simulink model "afe_dq_ttype"  (R2026b)
settings: Solver=ode23tb  StopTime=param.sim.simlength  FixedStep=param.sim.tc  MaxStep=param.glb_time.tc
values from neighbouring files (symbols this model uses):
  param = struct()    [init_model.m]
undefined symbols (not defined in the file or in its folder): magnitude
libraries: fl_lib x281, nesl_utility x136, igbt_simple_2th_lib x12, single_phase_transformer_lib x3, discrete_time_low_pass_filter x1, threephase_inductor_lib x1, dclink_for_three_levels x1, three_phase_three_level_ttype_inverter_ideal_switch_based_model x1, three_phase_three_levels_PWM_modulator x1, three_phase_bridge_three_level_ttype_igbt_simple_2th x1, three_phase_voltage_with_frt_emulator_mfcn x1
(part 4 of 8)

== system afe_dq_ttype/afe_dq_mod1/afe/deadtime_generator_for_ttype/dead_time_generator_cmos_simulink_phv/dead_time_leg_generator_1 ==
  cmd_in_QA : Inport
  cmd_in_QB : Inport  Port=2
  MATLAB Function : MATLAB Function  TreatAsAtomicUnit=on
  MATLAB Function1 : MATLAB Function  TreatAsAtomicUnit=on
  MATLAB Function2 : MATLAB Function  TreatAsAtomicUnit=on
  MATLAB Function3 : MATLAB Function  TreatAsAtomicUnit=on
  MATLAB Function4 : MATLAB Function  TreatAsAtomicUnit=on
  MATLAB Function5 : MATLAB Function  TreatAsAtomicUnit=on
  MATLAB Function6 : MATLAB Function  TreatAsAtomicUnit=on
  MATLAB Function7 : MATLAB Function  TreatAsAtomicUnit=on
  MATLAB Function8 : MATLAB Function  TreatAsAtomicUnit=on
  MATLAB Function9 : MATLAB Function  TreatAsAtomicUnit=on
  Transfer Fcn : TransferFcn  Denominator=[sqrt(2)*deadtime 1]
  Transfer Fcn1 : TransferFcn  Denominator=[sqrt(2)*deadtime 1]
  cmd_out_QA : Outport
  cmd_out_QB : Outport  Port=2
  wires:
  Transfer Fcn/1 -> MATLAB Function3/1(u)
  Transfer Fcn1/1 -> MATLAB Function8/1(u)
  cmd_in_QB/1 -> MATLAB Function6/1(u)
  MATLAB Function1/1(y) -> MATLAB Function9/1(u1)
  MATLAB Function5/1(y) -> MATLAB Function4/2(u2)
  cmd_in_QA/1 -> MATLAB Function/1(u)
  MATLAB Function6/1(y) -> MATLAB Function7/1(u), MATLAB Function5/1(u1)
  MATLAB Function4/1(y) -> cmd_out_QA/1
  MATLAB Function9/1(y) -> cmd_out_QB/1
  MATLAB Function/1(y) -> MATLAB Function2/1(u), MATLAB Function1/1(u1)
  MATLAB Function2/1(y) -> MATLAB Function4/1(u1), Transfer Fcn/1
  MATLAB Function3/1(y) -> MATLAB Function1/2(u2)
  MATLAB Function7/1(y) -> MATLAB Function9/2(u2), Transfer Fcn1/1
  MATLAB Function8/1(y) -> MATLAB Function5/2(u2)

== system afe_dq_ttype/afe_dq_mod1/afe/deadtime_generator_for_ttype/dead_time_generator_cmos_simulink_phw/dead_time_leg_generator_1 ==
  cmd_in_QA : Inport
  cmd_in_QB : Inport  Port=2
  MATLAB Function : MATLAB Function  TreatAsAtomicUnit=on
  MATLAB Function1 : MATLAB Function  TreatAsAtomicUnit=on
  MATLAB Function2 : MATLAB Function  TreatAsAtomicUnit=on
  MATLAB Function3 : MATLAB Function  TreatAsAtomicUnit=on
  MATLAB Function4 : MATLAB Function  TreatAsAtomicUnit=on
  MATLAB Function5 : MATLAB Function  TreatAsAtomicUnit=on
  MATLAB Function6 : MATLAB Function  TreatAsAtomicUnit=on
  MATLAB Function7 : MATLAB Function  TreatAsAtomicUnit=on
  MATLAB Function8 : MATLAB Function  TreatAsAtomicUnit=on
  MATLAB Function9 : MATLAB Function  TreatAsAtomicUnit=on
  Transfer Fcn : TransferFcn  Denominator=[sqrt(2)*deadtime 1]
  Transfer Fcn1 : TransferFcn  Denominator=[sqrt(2)*deadtime 1]
  cmd_out_QA : Outport
  cmd_out_QB : Outport  Port=2
  wires:
  MATLAB Function8/1(y) -> MATLAB Function5/2(u2)
  MATLAB Function7/1(y) -> Transfer Fcn1/1, MATLAB Function9/2(u2)
  MATLAB Function3/1(y) -> MATLAB Function1/2(u2)
  MATLAB Function2/1(y) -> Transfer Fcn/1, MATLAB Function4/1(u1)
  MATLAB Function/1(y) -> MATLAB Function1/1(u1), MATLAB Function2/1(u)
  MATLAB Function9/1(y) -> cmd_out_QB/1
  MATLAB Function4/1(y) -> cmd_out_QA/1
  MATLAB Function6/1(y) -> MATLAB Function5/1(u1), MATLAB Function7/1(u)
  cmd_in_QA/1 -> MATLAB Function/1(u)
  MATLAB Function5/1(y) -> MATLAB Function4/2(u2)
  MATLAB Function1/1(y) -> MATLAB Function9/1(u1)
  cmd_in_QB/1 -> MATLAB Function6/1(u)
  Transfer Fcn1/1 -> MATLAB Function8/1(u)
  Transfer Fcn/1 -> MATLAB Function3/1(u)

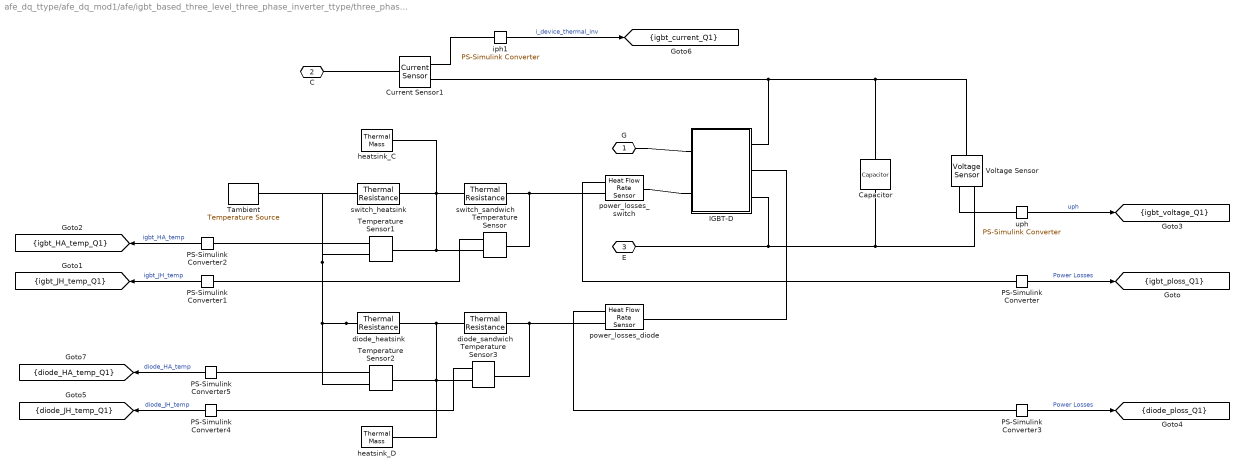
== system afe_dq_ttype/afe_dq_mod1/afe/igbt_based_three_level_three_phase_inverter_ttype/three_phase_inverter_igbt_2th_based_ttype/igbt_thermal_1 ==
  Capacitor : fl_lib/Electrical/Electrical Elements/Capacitor  c=Csnubber_m F  r=Rsnubber_m Ohm  g=0 1/Ohm  i_specify=off  i_priority=None  i=0 A  i_nominal_specify=off  i_nominal_value=1  i_nominal_unit=A  v_specify=off  v_priority=None  v=0 V  v_nominal_specify=off  v_nominal_value=1  v_nominal_unit=V  vc_specify=off  vc_priority=High  vc=0 V  vc_nominal_specify=off  vc_nominal_value=1  vc_nominal_unit=V
  Current Sensor1 : fl_lib/Electrical/Electrical Sensors/Current Sensor
  IGBT-D : Subsystem
  PS-Simulink Converter : nesl_utility/PS-Simulink Converter  PhysicalDomain=network_engine_domain  SubClassName=ps_output  LeftPortType=input  RightPortType=output  PseudoPeriodic=off  Frequencies=[]  VectorFormat=1-D array  Unit=W  AffineConversion=off
  PS-Simulink Converter{1..2,4..5} (4 alike) : nesl_utility/PS-Simulink Converter  PhysicalDomain=network_engine_domain  SubClassName=ps_output  LeftPortType=input  RightPortType=output  PseudoPeriodic=off  Frequencies=[]  VectorFormat=1-D array  Unit=degC  AffineConversion=off
  PS-Simulink Converter3 : nesl_utility/PS-Simulink Converter  PhysicalDomain=network_engine_domain  SubClassName=ps_output  LeftPortType=input  RightPortType=output  PseudoPeriodic=off  Frequencies=[]  VectorFormat=1-D array  Unit=W  AffineConversion=off
  Tambient : fl_lib/Thermal/Thermal Sources/Temperature Source  temperature=Tambient_m degC
  Temperature Sensor{,1..3} (4 alike) : fl_lib/Thermal/Thermal Sensors/Temperature Sensor  temperature_measure=foundation.enum.MeasurementReference.difference
  Voltage Sensor : fl_lib/Electrical/Electrical Sensors/Voltage Sensor
  diode_heatsink : fl_lib/Thermal/Thermal Elements/Thermal Resistance  resistance=rth_diode_HA_m K/W  T_specify=off  T_priority=High  T=0 deltadegC  T_nominal_specify=off  T_nominal_value=1  T_nominal_unit=K  Q_specify=off  Q_priority=None  Q=0 W  Q_nominal_specify=off  Q_nominal_value=1  Q_nominal_unit=W
  diode_sandwich : fl_lib/Thermal/Thermal Elements/Thermal Resistance  resistance=rth_diode_JH_m K/W  T_specify=off  T_priority=High  T=0 degC  T_nominal_specify=off  T_nominal_value=1  T_nominal_unit=K  Q_specify=off  Q_priority=None  Q=0 W  Q_nominal_specify=off  Q_nominal_value=1  Q_nominal_unit=W
  heatsink_C : fl_lib/Thermal/Thermal Elements/Thermal Mass  mass_type=foundation.enum.constant_variable.constant  mass=mass_heatsink_m kg  sp_heat=specific_heat_m J/(K*kg)  mass_min=1e-6 kg  num_ports=foundation.enum.numPorts2.one  m_specify=off  m_priority=High  m=1 kg  m_nominal_specify=off  m_nominal_value=1  m_nominal_unit=kg  T_specify=on  T_priority=High  T=DThs_init_m+Tambient_m degC  T_nominal_specify=off  T_nominal_value=1  T_nominal_unit=K  Q_specify=off  Q_priority=High  Q=0 W  Q_nominal_specify=off  Q_nominal_value=1  Q_nominal_unit=W
  heatsink_D : fl_lib/Thermal/Thermal Elements/Thermal Mass  mass_type=foundation.enum.constant_variable.constant  mass=mass_heatsink_m kg  sp_heat=specific_heat_m J/(K*kg)  mass_min=1e-6 kg  num_ports=foundation.enum.numPorts2.one  m_specify=off  m_priority=High  m=1 kg  m_nominal_specify=off  m_nominal_value=1  m_nominal_unit=kg  T_specify=on  T_priority=High  T=DThs_init_m+Tambient_m degC  T_nominal_specify=off  T_nominal_value=1  T_nominal_unit=K  Q_specify=off  Q_priority=High  Q=0 W  Q_nominal_specify=off  Q_nominal_value=1  Q_nominal_unit=W
  iph1 : nesl_utility/PS-Simulink Converter  PhysicalDomain=network_engine_domain  SubClassName=ps_output  LeftPortType=input  RightPortType=output  PseudoPeriodic=off  Frequencies=[]  VectorFormat=1-D array  Unit=A  AffineConversion=off
  power_losses_diode : fl_lib/Thermal/Thermal Sensors/Heat Flow Rate Sensor
  power_losses_switch : fl_lib/Thermal/Thermal Sensors/Heat Flow Rate Sensor
  switch_heatsink : fl_lib/Thermal/Thermal Elements/Thermal Resistance  resistance=rth_switch_HA_m K/W  T_specify=off  T_priority=High  T=0 deltadegC  T_nominal_specify=off  T_nominal_value=1  T_nominal_unit=K  Q_specify=off  Q_priority=None  Q=0 W  Q_nominal_specify=off  Q_nominal_value=1  Q_nominal_unit=W
  switch_sandwich : fl_lib/Thermal/Thermal Elements/Thermal Resistance  resistance=rth_switch_JH_m K/W  T_specify=off  T_priority=High  T=0 degC  T_nominal_specify=off  T_nominal_value=1  T_nominal_unit=K  Q_specify=off  Q_priority=None  Q=0 W  Q_nominal_specify=off  Q_nominal_value=1  Q_nominal_unit=W
  uph : nesl_utility/PS-Simulink Converter  PhysicalDomain=network_engine_domain  SubClassName=ps_output  LeftPortType=input  RightPortType=output  PseudoPeriodic=off  Frequencies=[]  VectorFormat=1-D array  Unit=V  AffineConversion=off
  G : PMIOPort  Side=Left
  C : PMIOPort  Port=2  Side=Left
  E : PMIOPort  Port=3  Side=Right
  tag scope: diode_HA_temp_Q1=scoped, diode_JH_temp_Q1=scoped, diode_ploss_Q1=scoped, igbt_HA_temp_Q1=scoped, igbt_JH_temp_Q1=scoped, igbt_current_Q1=scoped, igbt_ploss_Q1=scoped, igbt_voltage_Q1=scoped
  wires:
  PS-Simulink Converter/1 -> [igbt_ploss_Q1]  "Power Losses"
  PS-Simulink Converter2/1 -> [igbt_HA_temp_Q1]  "igbt_HA_temp"
  PS-Simulink Converter1/1 -> [igbt_JH_temp_Q1]  "igbt_JH_temp"
  iph1/1 -> [igbt_current_Q1]  "i_device_thermal_inv"
  uph/1 -> [igbt_voltage_Q1]  "uph"
  PS-Simulink Converter3/1 -> [diode_ploss_Q1]  "Power Losses"
  PS-Simulink Converter4/1 -> [diode_JH_temp_Q1]  "diode_JH_temp"
  PS-Simulink Converter5/1 -> [diode_HA_temp_Q1]  "diode_HA_temp"
  connections:
  Voltage Sensor/RConn2 -- Capacitor/RConn1 -- E/RConn1 -- IGBT-D/RConn3
  PS-Simulink Converter/LConn1 -- power_losses_switch/RConn1
  Temperature Sensor/LConn1 -- power_losses_switch/RConn2 -- switch_sandwich/LConn1
  Temperature Sensor1/LConn1 -- Temperature Sensor/RConn1 -- switch_sandwich/RConn1 -- switch_heatsink/LConn1 -- heatsink_C/LConn1
  Temperature Sensor/RConn2 -- PS-Simulink Converter1/LConn1
  diode_heatsink/RConn1 -- Temperature Sensor2/RConn1 -- Temperature Sensor1/RConn1 -- Tambient/LConn1 -- switch_heatsink/RConn1
  Temperature Sensor1/RConn2 -- PS-Simulink Converter2/LConn1
  Current Sensor1/LConn1 -- C/RConn1
  Capacitor/LConn1 -- Voltage Sensor/LConn1 -- Current Sensor1/RConn2 -- IGBT-D/RConn1
  Current Sensor1/RConn1 -- iph1/LConn1
  Voltage Sensor/RConn1 -- uph/LConn1
  power_losses_diode/RConn2 -- Temperature Sensor3/LConn1 -- diode_sandwich/LConn1
  heatsink_D/LConn1 -- Temperature Sensor2/LConn1 -- Temperature Sensor3/RConn1 -- diode_sandwich/RConn1 -- diode_heatsink/LConn1
  power_losses_diode/RConn1 -- PS-Simulink Converter3/LConn1
  Temperature Sensor2/RConn2 -- PS-Simulink Converter5/LConn1
  Temperature Sensor3/RConn2 -- PS-Simulink Converter4/LConn1
  IGBT-D/LConn2 -- power_losses_switch/LConn1
  G/RConn1 -- IGBT-D/LConn1
  IGBT-D/RConn2 -- power_losses_diode/LConn1

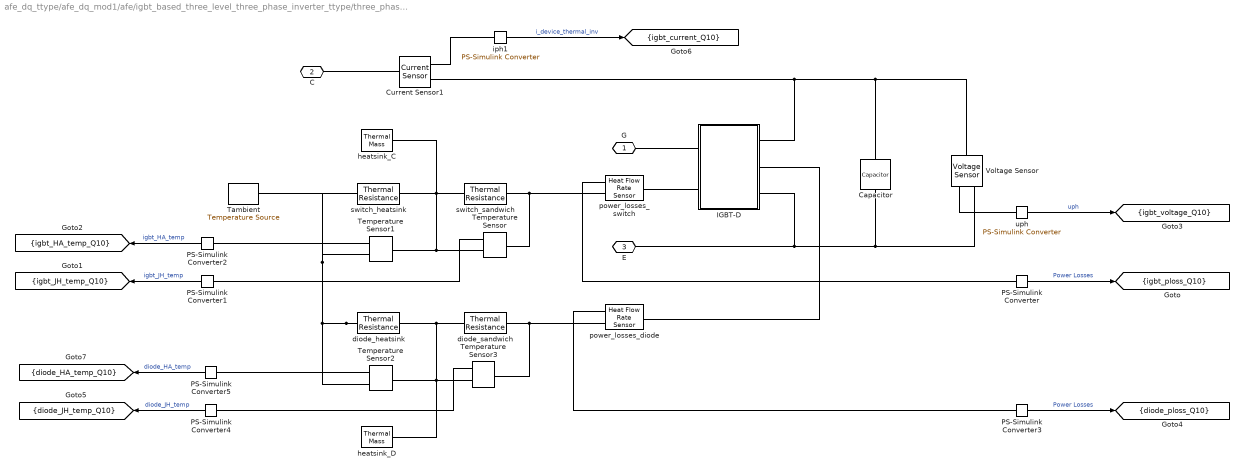
== system afe_dq_ttype/afe_dq_mod1/afe/igbt_based_three_level_three_phase_inverter_ttype/three_phase_inverter_igbt_2th_based_ttype/igbt_thermal_10 ==
  Capacitor : fl_lib/Electrical/Electrical Elements/Capacitor  c=Csnubber_m F  r=Rsnubber_m Ohm  g=0 1/Ohm  i_specify=off  i_priority=None  i=0 A  i_nominal_specify=off  i_nominal_value=1  i_nominal_unit=A  v_specify=off  v_priority=None  v=0 V  v_nominal_specify=off  v_nominal_value=1  v_nominal_unit=V  vc_specify=off  vc_priority=High  vc=0 V  vc_nominal_specify=off  vc_nominal_value=1  vc_nominal_unit=V
  Current Sensor1 : fl_lib/Electrical/Electrical Sensors/Current Sensor
  IGBT-D : Subsystem
  PS-Simulink Converter : nesl_utility/PS-Simulink Converter  PhysicalDomain=network_engine_domain  SubClassName=ps_output  LeftPortType=input  RightPortType=output  PseudoPeriodic=off  Frequencies=[]  VectorFormat=1-D array  Unit=W  AffineConversion=off
  PS-Simulink Converter{1..2,4..5} (4 alike) : nesl_utility/PS-Simulink Converter  PhysicalDomain=network_engine_domain  SubClassName=ps_output  LeftPortType=input  RightPortType=output  PseudoPeriodic=off  Frequencies=[]  VectorFormat=1-D array  Unit=degC  AffineConversion=off
  PS-Simulink Converter3 : nesl_utility/PS-Simulink Converter  PhysicalDomain=network_engine_domain  SubClassName=ps_output  LeftPortType=input  RightPortType=output  PseudoPeriodic=off  Frequencies=[]  VectorFormat=1-D array  Unit=W  AffineConversion=off
  Tambient : fl_lib/Thermal/Thermal Sources/Temperature Source  temperature=Tambient_m degC
  Temperature Sensor{,1..3} (4 alike) : fl_lib/Thermal/Thermal Sensors/Temperature Sensor  temperature_measure=foundation.enum.MeasurementReference.difference
  Voltage Sensor : fl_lib/Electrical/Electrical Sensors/Voltage Sensor
  diode_heatsink : fl_lib/Thermal/Thermal Elements/Thermal Resistance  resistance=rth_diode_HA_m K/W  T_specify=off  T_priority=High  T=0 deltadegC  T_nominal_specify=off  T_nominal_value=1  T_nominal_unit=K  Q_specify=off  Q_priority=None  Q=0 W  Q_nominal_specify=off  Q_nominal_value=1  Q_nominal_unit=W
  diode_sandwich : fl_lib/Thermal/Thermal Elements/Thermal Resistance  resistance=rth_diode_JH_m K/W  T_specify=off  T_priority=High  T=0 degC  T_nominal_specify=off  T_nominal_value=1  T_nominal_unit=K  Q_specify=off  Q_priority=None  Q=0 W  Q_nominal_specify=off  Q_nominal_value=1  Q_nominal_unit=W
  heatsink_C : fl_lib/Thermal/Thermal Elements/Thermal Mass  mass_type=foundation.enum.constant_variable.constant  mass=mass_heatsink_m kg  sp_heat=specific_heat_m J/(K*kg)  mass_min=1e-6 kg  num_ports=foundation.enum.numPorts2.one  m_specify=off  m_priority=High  m=1 kg  m_nominal_specify=off  m_nominal_value=1  m_nominal_unit=kg  T_specify=on  T_priority=High  T=DThs_init_m+Tambient_m degC  T_nominal_specify=off  T_nominal_value=1  T_nominal_unit=K  Q_specify=off  Q_priority=High  Q=0 W  Q_nominal_specify=off  Q_nominal_value=1  Q_nominal_unit=W
  heatsink_D : fl_lib/Thermal/Thermal Elements/Thermal Mass  mass_type=foundation.enum.constant_variable.constant  mass=mass_heatsink_m kg  sp_heat=specific_heat_m J/(K*kg)  mass_min=1e-6 kg  num_ports=foundation.enum.numPorts2.one  m_specify=off  m_priority=High  m=1 kg  m_nominal_specify=off  m_nominal_value=1  m_nominal_unit=kg  T_specify=on  T_priority=High  T=DThs_init_m+Tambient_m degC  T_nominal_specify=off  T_nominal_value=1  T_nominal_unit=K  Q_specify=off  Q_priority=High  Q=0 W  Q_nominal_specify=off  Q_nominal_value=1  Q_nominal_unit=W
  iph1 : nesl_utility/PS-Simulink Converter  PhysicalDomain=network_engine_domain  SubClassName=ps_output  LeftPortType=input  RightPortType=output  PseudoPeriodic=off  Frequencies=[]  VectorFormat=1-D array  Unit=A  AffineConversion=off
  power_losses_diode : fl_lib/Thermal/Thermal Sensors/Heat Flow Rate Sensor
  power_losses_switch : fl_lib/Thermal/Thermal Sensors/Heat Flow Rate Sensor
  switch_heatsink : fl_lib/Thermal/Thermal Elements/Thermal Resistance  resistance=rth_switch_HA_m K/W  T_specify=off  T_priority=High  T=0 deltadegC  T_nominal_specify=off  T_nominal_value=1  T_nominal_unit=K  Q_specify=off  Q_priority=None  Q=0 W  Q_nominal_specify=off  Q_nominal_value=1  Q_nominal_unit=W
  switch_sandwich : fl_lib/Thermal/Thermal Elements/Thermal Resistance  resistance=rth_switch_JH_m K/W  T_specify=off  T_priority=High  T=0 degC  T_nominal_specify=off  T_nominal_value=1  T_nominal_unit=K  Q_specify=off  Q_priority=None  Q=0 W  Q_nominal_specify=off  Q_nominal_value=1  Q_nominal_unit=W
  uph : nesl_utility/PS-Simulink Converter  PhysicalDomain=network_engine_domain  SubClassName=ps_output  LeftPortType=input  RightPortType=output  PseudoPeriodic=off  Frequencies=[]  VectorFormat=1-D array  Unit=V  AffineConversion=off
  G : PMIOPort  Side=Left
  C : PMIOPort  Port=2  Side=Left
  E : PMIOPort  Port=3  Side=Right
  tag scope: diode_HA_temp_Q10=scoped, diode_JH_temp_Q10=scoped, diode_ploss_Q10=scoped, igbt_HA_temp_Q10=scoped, igbt_JH_temp_Q10=scoped, igbt_current_Q10=scoped, igbt_ploss_Q10=scoped, igbt_voltage_Q10=scoped
  wires:
  PS-Simulink Converter/1 -> [igbt_ploss_Q10]  "Power Losses"
  PS-Simulink Converter2/1 -> [igbt_HA_temp_Q10]  "igbt_HA_temp"
  PS-Simulink Converter1/1 -> [igbt_JH_temp_Q10]  "igbt_JH_temp"
  iph1/1 -> [igbt_current_Q10]  "i_device_thermal_inv"
  uph/1 -> [igbt_voltage_Q10]  "uph"
  PS-Simulink Converter3/1 -> [diode_ploss_Q10]  "Power Losses"
  PS-Simulink Converter4/1 -> [diode_JH_temp_Q10]  "diode_JH_temp"
  PS-Simulink Converter5/1 -> [diode_HA_temp_Q10]  "diode_HA_temp"
  connections:
  Voltage Sensor/RConn2 -- Capacitor/RConn1 -- IGBT-D/RConn3 -- E/RConn1
  PS-Simulink Converter/LConn1 -- power_losses_switch/RConn1
  Temperature Sensor/LConn1 -- power_losses_switch/RConn2 -- switch_sandwich/LConn1
  Temperature Sensor1/LConn1 -- Temperature Sensor/RConn1 -- switch_sandwich/RConn1 -- switch_heatsink/LConn1 -- heatsink_C/LConn1
  Temperature Sensor/RConn2 -- PS-Simulink Converter1/LConn1
  diode_heatsink/RConn1 -- Temperature Sensor2/RConn1 -- Temperature Sensor1/RConn1 -- Tambient/LConn1 -- switch_heatsink/RConn1
  Temperature Sensor1/RConn2 -- PS-Simulink Converter2/LConn1
  Current Sensor1/LConn1 -- C/RConn1
  Capacitor/LConn1 -- Voltage Sensor/LConn1 -- IGBT-D/RConn1 -- Current Sensor1/RConn2
  Current Sensor1/RConn1 -- iph1/LConn1
  Voltage Sensor/RConn1 -- uph/LConn1
  power_losses_diode/RConn2 -- Temperature Sensor3/LConn1 -- diode_sandwich/LConn1
  heatsink_D/LConn1 -- Temperature Sensor2/LConn1 -- Temperature Sensor3/RConn1 -- diode_sandwich/RConn1 -- diode_heatsink/LConn1
  power_losses_diode/RConn1 -- PS-Simulink Converter3/LConn1
  Temperature Sensor2/RConn2 -- PS-Simulink Converter5/LConn1
  Temperature Sensor3/RConn2 -- PS-Simulink Converter4/LConn1
  IGBT-D/LConn2 -- power_losses_switch/LConn1
  G/RConn1 -- IGBT-D/LConn1
  IGBT-D/RConn2 -- power_losses_diode/LConn1

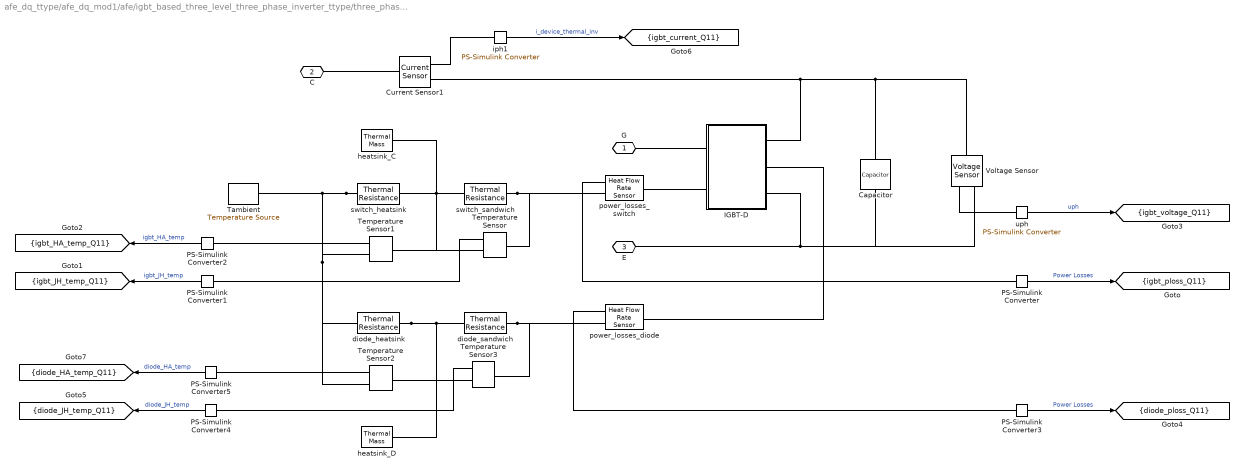
== system afe_dq_ttype/afe_dq_mod1/afe/igbt_based_three_level_three_phase_inverter_ttype/three_phase_inverter_igbt_2th_based_ttype/igbt_thermal_11 ==
  Capacitor : fl_lib/Electrical/Electrical Elements/Capacitor  c=Csnubber_m F  r=Rsnubber_m Ohm  g=0 1/Ohm  i_specify=off  i_priority=None  i=0 A  i_nominal_specify=off  i_nominal_value=1  i_nominal_unit=A  v_specify=off  v_priority=None  v=0 V  v_nominal_specify=off  v_nominal_value=1  v_nominal_unit=V  vc_specify=off  vc_priority=High  vc=0 V  vc_nominal_specify=off  vc_nominal_value=1  vc_nominal_unit=V
  Current Sensor1 : fl_lib/Electrical/Electrical Sensors/Current Sensor
  IGBT-D : Subsystem
  PS-Simulink Converter : nesl_utility/PS-Simulink Converter  PhysicalDomain=network_engine_domain  SubClassName=ps_output  LeftPortType=input  RightPortType=output  PseudoPeriodic=off  Frequencies=[]  VectorFormat=1-D array  Unit=W  AffineConversion=off
  PS-Simulink Converter{1..2,4..5} (4 alike) : nesl_utility/PS-Simulink Converter  PhysicalDomain=network_engine_domain  SubClassName=ps_output  LeftPortType=input  RightPortType=output  PseudoPeriodic=off  Frequencies=[]  VectorFormat=1-D array  Unit=degC  AffineConversion=off
  PS-Simulink Converter3 : nesl_utility/PS-Simulink Converter  PhysicalDomain=network_engine_domain  SubClassName=ps_output  LeftPortType=input  RightPortType=output  PseudoPeriodic=off  Frequencies=[]  VectorFormat=1-D array  Unit=W  AffineConversion=off
  Tambient : fl_lib/Thermal/Thermal Sources/Temperature Source  temperature=Tambient_m degC
  Temperature Sensor{,1..3} (4 alike) : fl_lib/Thermal/Thermal Sensors/Temperature Sensor  temperature_measure=foundation.enum.MeasurementReference.difference
  Voltage Sensor : fl_lib/Electrical/Electrical Sensors/Voltage Sensor
  diode_heatsink : fl_lib/Thermal/Thermal Elements/Thermal Resistance  resistance=rth_diode_HA_m K/W  T_specify=off  T_priority=High  T=0 deltadegC  T_nominal_specify=off  T_nominal_value=1  T_nominal_unit=K  Q_specify=off  Q_priority=None  Q=0 W  Q_nominal_specify=off  Q_nominal_value=1  Q_nominal_unit=W
  diode_sandwich : fl_lib/Thermal/Thermal Elements/Thermal Resistance  resistance=rth_diode_JH_m K/W  T_specify=off  T_priority=High  T=0 degC  T_nominal_specify=off  T_nominal_value=1  T_nominal_unit=K  Q_specify=off  Q_priority=None  Q=0 W  Q_nominal_specify=off  Q_nominal_value=1  Q_nominal_unit=W
  heatsink_C : fl_lib/Thermal/Thermal Elements/Thermal Mass  mass_type=foundation.enum.constant_variable.constant  mass=mass_heatsink_m kg  sp_heat=specific_heat_m J/(K*kg)  mass_min=1e-6 kg  num_ports=foundation.enum.numPorts2.one  m_specify=off  m_priority=High  m=1 kg  m_nominal_specify=off  m_nominal_value=1  m_nominal_unit=kg  T_specify=on  T_priority=High  T=DThs_init_m+Tambient_m degC  T_nominal_specify=off  T_nominal_value=1  T_nominal_unit=K  Q_specify=off  Q_priority=High  Q=0 W  Q_nominal_specify=off  Q_nominal_value=1  Q_nominal_unit=W
  heatsink_D : fl_lib/Thermal/Thermal Elements/Thermal Mass  mass_type=foundation.enum.constant_variable.constant  mass=mass_heatsink_m kg  sp_heat=specific_heat_m J/(K*kg)  mass_min=1e-6 kg  num_ports=foundation.enum.numPorts2.one  m_specify=off  m_priority=High  m=1 kg  m_nominal_specify=off  m_nominal_value=1  m_nominal_unit=kg  T_specify=on  T_priority=High  T=DThs_init_m+Tambient_m degC  T_nominal_specify=off  T_nominal_value=1  T_nominal_unit=K  Q_specify=off  Q_priority=High  Q=0 W  Q_nominal_specify=off  Q_nominal_value=1  Q_nominal_unit=W
  iph1 : nesl_utility/PS-Simulink Converter  PhysicalDomain=network_engine_domain  SubClassName=ps_output  LeftPortType=input  RightPortType=output  PseudoPeriodic=off  Frequencies=[]  VectorFormat=1-D array  Unit=A  AffineConversion=off
  power_losses_diode : fl_lib/Thermal/Thermal Sensors/Heat Flow Rate Sensor
  power_losses_switch : fl_lib/Thermal/Thermal Sensors/Heat Flow Rate Sensor
  switch_heatsink : fl_lib/Thermal/Thermal Elements/Thermal Resistance  resistance=rth_switch_HA_m K/W  T_specify=off  T_priority=High  T=0 deltadegC  T_nominal_specify=off  T_nominal_value=1  T_nominal_unit=K  Q_specify=off  Q_priority=None  Q=0 W  Q_nominal_specify=off  Q_nominal_value=1  Q_nominal_unit=W
  switch_sandwich : fl_lib/Thermal/Thermal Elements/Thermal Resistance  resistance=rth_switch_JH_m K/W  T_specify=off  T_priority=High  T=0 degC  T_nominal_specify=off  T_nominal_value=1  T_nominal_unit=K  Q_specify=off  Q_priority=None  Q=0 W  Q_nominal_specify=off  Q_nominal_value=1  Q_nominal_unit=W
  uph : nesl_utility/PS-Simulink Converter  PhysicalDomain=network_engine_domain  SubClassName=ps_output  LeftPortType=input  RightPortType=output  PseudoPeriodic=off  Frequencies=[]  VectorFormat=1-D array  Unit=V  AffineConversion=off
  G : PMIOPort  Side=Left
  C : PMIOPort  Port=2  Side=Left
  E : PMIOPort  Port=3  Side=Right
  tag scope: diode_HA_temp_Q11=scoped, diode_JH_temp_Q11=scoped, diode_ploss_Q11=scoped, igbt_HA_temp_Q11=scoped, igbt_JH_temp_Q11=scoped, igbt_current_Q11=scoped, igbt_ploss_Q11=scoped, igbt_voltage_Q11=scoped
  wires:
  PS-Simulink Converter5/1 -> [diode_HA_temp_Q11]  "diode_HA_temp"
  PS-Simulink Converter4/1 -> [diode_JH_temp_Q11]  "diode_JH_temp"
  PS-Simulink Converter3/1 -> [diode_ploss_Q11]  "Power Losses"
  uph/1 -> [igbt_voltage_Q11]  "uph"
  iph1/1 -> [igbt_current_Q11]  "i_device_thermal_inv"
  PS-Simulink Converter1/1 -> [igbt_JH_temp_Q11]  "igbt_JH_temp"
  PS-Simulink Converter2/1 -> [igbt_HA_temp_Q11]  "igbt_HA_temp"
  PS-Simulink Converter/1 -> [igbt_ploss_Q11]  "Power Losses"
  connections:
  Temperature Sensor3/RConn2 -- PS-Simulink Converter4/LConn1
  Temperature Sensor2/RConn2 -- PS-Simulink Converter5/LConn1
  power_losses_diode/RConn1 -- PS-Simulink Converter3/LConn1
  diode_heatsink/LConn1 -- diode_sandwich/RConn1 -- Temperature Sensor3/RConn1 -- Temperature Sensor2/LConn1 -- heatsink_D/LConn1
  diode_sandwich/LConn1 -- Temperature Sensor3/LConn1 -- power_losses_diode/RConn2
  Voltage Sensor/RConn1 -- uph/LConn1
  Current Sensor1/RConn1 -- iph1/LConn1
  Current Sensor1/RConn2 -- IGBT-D/RConn1 -- Voltage Sensor/LConn1 -- Capacitor/LConn1
  Current Sensor1/LConn1 -- C/RConn1
  Temperature Sensor1/RConn2 -- PS-Simulink Converter2/LConn1
  switch_heatsink/RConn1 -- Tambient/LConn1 -- Temperature Sensor1/RConn1 -- Temperature Sensor2/RConn1 -- diode_heatsink/RConn1
  Temperature Sensor/RConn2 -- PS-Simulink Converter1/LConn1
  heatsink_C/LConn1 -- switch_heatsink/LConn1 -- switch_sandwich/RConn1 -- Temperature Sensor/RConn1 -- Temperature Sensor1/LConn1
  switch_sandwich/LConn1 -- power_losses_switch/RConn2 -- Temperature Sensor/LConn1
  PS-Simulink Converter/LConn1 -- power_losses_switch/RConn1
  Capacitor/RConn1 -- Voltage Sensor/RConn2 -- IGBT-D/RConn3 -- E/RConn1
  IGBT-D/LConn2 -- power_losses_switch/LConn1
  G/RConn1 -- IGBT-D/LConn1
  IGBT-D/RConn2 -- power_losses_diode/LConn1

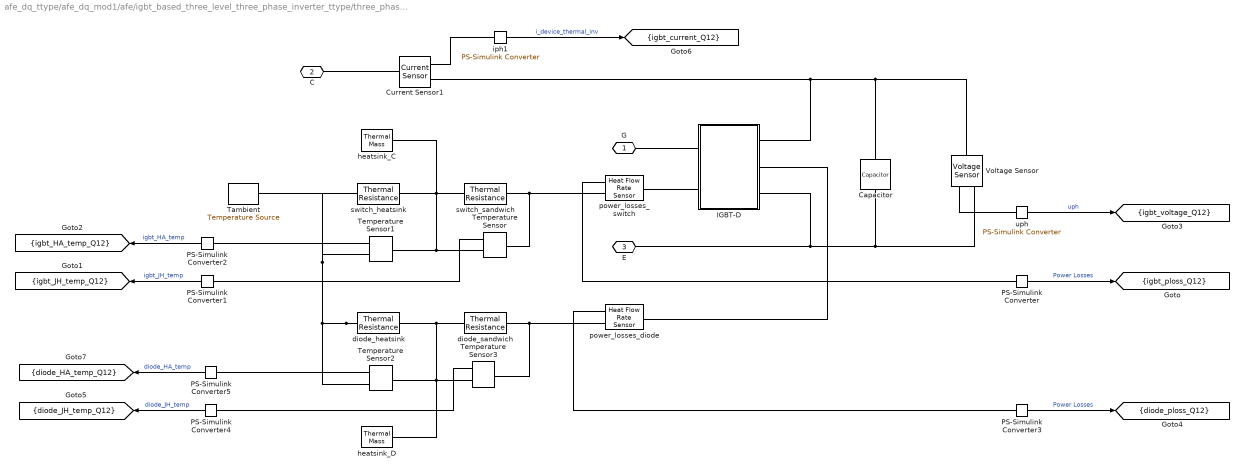
== system afe_dq_ttype/afe_dq_mod1/afe/igbt_based_three_level_three_phase_inverter_ttype/three_phase_inverter_igbt_2th_based_ttype/igbt_thermal_12 ==
  Capacitor : fl_lib/Electrical/Electrical Elements/Capacitor  c=Csnubber_m F  r=Rsnubber_m Ohm  g=0 1/Ohm  i_specify=off  i_priority=None  i=0 A  i_nominal_specify=off  i_nominal_value=1  i_nominal_unit=A  v_specify=off  v_priority=None  v=0 V  v_nominal_specify=off  v_nominal_value=1  v_nominal_unit=V  vc_specify=off  vc_priority=High  vc=0 V  vc_nominal_specify=off  vc_nominal_value=1  vc_nominal_unit=V
  Current Sensor1 : fl_lib/Electrical/Electrical Sensors/Current Sensor
  IGBT-D : Subsystem
  PS-Simulink Converter : nesl_utility/PS-Simulink Converter  PhysicalDomain=network_engine_domain  SubClassName=ps_output  LeftPortType=input  RightPortType=output  PseudoPeriodic=off  Frequencies=[]  VectorFormat=1-D array  Unit=W  AffineConversion=off
  PS-Simulink Converter{1..2,4..5} (4 alike) : nesl_utility/PS-Simulink Converter  PhysicalDomain=network_engine_domain  SubClassName=ps_output  LeftPortType=input  RightPortType=output  PseudoPeriodic=off  Frequencies=[]  VectorFormat=1-D array  Unit=degC  AffineConversion=off
  PS-Simulink Converter3 : nesl_utility/PS-Simulink Converter  PhysicalDomain=network_engine_domain  SubClassName=ps_output  LeftPortType=input  RightPortType=output  PseudoPeriodic=off  Frequencies=[]  VectorFormat=1-D array  Unit=W  AffineConversion=off
  Tambient : fl_lib/Thermal/Thermal Sources/Temperature Source  temperature=Tambient_m degC
  Temperature Sensor{,1..3} (4 alike) : fl_lib/Thermal/Thermal Sensors/Temperature Sensor  temperature_measure=foundation.enum.MeasurementReference.difference
  Voltage Sensor : fl_lib/Electrical/Electrical Sensors/Voltage Sensor
  diode_heatsink : fl_lib/Thermal/Thermal Elements/Thermal Resistance  resistance=rth_diode_HA_m K/W  T_specify=off  T_priority=High  T=0 deltadegC  T_nominal_specify=off  T_nominal_value=1  T_nominal_unit=K  Q_specify=off  Q_priority=None  Q=0 W  Q_nominal_specify=off  Q_nominal_value=1  Q_nominal_unit=W
  diode_sandwich : fl_lib/Thermal/Thermal Elements/Thermal Resistance  resistance=rth_diode_JH_m K/W  T_specify=off  T_priority=High  T=0 degC  T_nominal_specify=off  T_nominal_value=1  T_nominal_unit=K  Q_specify=off  Q_priority=None  Q=0 W  Q_nominal_specify=off  Q_nominal_value=1  Q_nominal_unit=W
  heatsink_C : fl_lib/Thermal/Thermal Elements/Thermal Mass  mass_type=foundation.enum.constant_variable.constant  mass=mass_heatsink_m kg  sp_heat=specific_heat_m J/(K*kg)  mass_min=1e-6 kg  num_ports=foundation.enum.numPorts2.one  m_specify=off  m_priority=High  m=1 kg  m_nominal_specify=off  m_nominal_value=1  m_nominal_unit=kg  T_specify=on  T_priority=High  T=DThs_init_m+Tambient_m degC  T_nominal_specify=off  T_nominal_value=1  T_nominal_unit=K  Q_specify=off  Q_priority=High  Q=0 W  Q_nominal_specify=off  Q_nominal_value=1  Q_nominal_unit=W
  heatsink_D : fl_lib/Thermal/Thermal Elements/Thermal Mass  mass_type=foundation.enum.constant_variable.constant  mass=mass_heatsink_m kg  sp_heat=specific_heat_m J/(K*kg)  mass_min=1e-6 kg  num_ports=foundation.enum.numPorts2.one  m_specify=off  m_priority=High  m=1 kg  m_nominal_specify=off  m_nominal_value=1  m_nominal_unit=kg  T_specify=on  T_priority=High  T=DThs_init_m+Tambient_m degC  T_nominal_specify=off  T_nominal_value=1  T_nominal_unit=K  Q_specify=off  Q_priority=High  Q=0 W  Q_nominal_specify=off  Q_nominal_value=1  Q_nominal_unit=W
  iph1 : nesl_utility/PS-Simulink Converter  PhysicalDomain=network_engine_domain  SubClassName=ps_output  LeftPortType=input  RightPortType=output  PseudoPeriodic=off  Frequencies=[]  VectorFormat=1-D array  Unit=A  AffineConversion=off
  power_losses_diode : fl_lib/Thermal/Thermal Sensors/Heat Flow Rate Sensor
  power_losses_switch : fl_lib/Thermal/Thermal Sensors/Heat Flow Rate Sensor
  switch_heatsink : fl_lib/Thermal/Thermal Elements/Thermal Resistance  resistance=rth_switch_HA_m K/W  T_specify=off  T_priority=High  T=0 deltadegC  T_nominal_specify=off  T_nominal_value=1  T_nominal_unit=K  Q_specify=off  Q_priority=None  Q=0 W  Q_nominal_specify=off  Q_nominal_value=1  Q_nominal_unit=W
  switch_sandwich : fl_lib/Thermal/Thermal Elements/Thermal Resistance  resistance=rth_switch_JH_m K/W  T_specify=off  T_priority=High  T=0 degC  T_nominal_specify=off  T_nominal_value=1  T_nominal_unit=K  Q_specify=off  Q_priority=None  Q=0 W  Q_nominal_specify=off  Q_nominal_value=1  Q_nominal_unit=W
  uph : nesl_utility/PS-Simulink Converter  PhysicalDomain=network_engine_domain  SubClassName=ps_output  LeftPortType=input  RightPortType=output  PseudoPeriodic=off  Frequencies=[]  VectorFormat=1-D array  Unit=V  AffineConversion=off
  G : PMIOPort  Side=Left
  C : PMIOPort  Port=2  Side=Left
  E : PMIOPort  Port=3  Side=Right
  tag scope: diode_HA_temp_Q12=scoped, diode_JH_temp_Q12=scoped, diode_ploss_Q12=scoped, igbt_HA_temp_Q12=scoped, igbt_JH_temp_Q12=scoped, igbt_current_Q12=scoped, igbt_ploss_Q12=scoped, igbt_voltage_Q12=scoped
  wires:
  PS-Simulink Converter/1 -> [igbt_ploss_Q12]  "Power Losses"
  PS-Simulink Converter2/1 -> [igbt_HA_temp_Q12]  "igbt_HA_temp"
  PS-Simulink Converter1/1 -> [igbt_JH_temp_Q12]  "igbt_JH_temp"
  iph1/1 -> [igbt_current_Q12]  "i_device_thermal_inv"
  uph/1 -> [igbt_voltage_Q12]  "uph"
  PS-Simulink Converter3/1 -> [diode_ploss_Q12]  "Power Losses"
  PS-Simulink Converter4/1 -> [diode_JH_temp_Q12]  "diode_JH_temp"
  PS-Simulink Converter5/1 -> [diode_HA_temp_Q12]  "diode_HA_temp"
  connections:
  Voltage Sensor/RConn2 -- Capacitor/RConn1 -- IGBT-D/RConn3 -- E/RConn1
  PS-Simulink Converter/LConn1 -- power_losses_switch/RConn1
  Temperature Sensor/LConn1 -- power_losses_switch/RConn2 -- switch_sandwich/LConn1
  Temperature Sensor1/LConn1 -- Temperature Sensor/RConn1 -- switch_sandwich/RConn1 -- switch_heatsink/LConn1 -- heatsink_C/LConn1
  Temperature Sensor/RConn2 -- PS-Simulink Converter1/LConn1
  diode_heatsink/RConn1 -- Temperature Sensor2/RConn1 -- Temperature Sensor1/RConn1 -- Tambient/LConn1 -- switch_heatsink/RConn1
  Temperature Sensor1/RConn2 -- PS-Simulink Converter2/LConn1
  Current Sensor1/LConn1 -- C/RConn1
  Capacitor/LConn1 -- Voltage Sensor/LConn1 -- IGBT-D/RConn1 -- Current Sensor1/RConn2
  Current Sensor1/RConn1 -- iph1/LConn1
  Voltage Sensor/RConn1 -- uph/LConn1
  power_losses_diode/RConn2 -- Temperature Sensor3/LConn1 -- diode_sandwich/LConn1
  heatsink_D/LConn1 -- Temperature Sensor2/LConn1 -- Temperature Sensor3/RConn1 -- diode_sandwich/RConn1 -- diode_heatsink/LConn1
  power_losses_diode/RConn1 -- PS-Simulink Converter3/LConn1
  Temperature Sensor2/RConn2 -- PS-Simulink Converter5/LConn1
  Temperature Sensor3/RConn2 -- PS-Simulink Converter4/LConn1
  IGBT-D/LConn2 -- power_losses_switch/LConn1
  G/RConn1 -- IGBT-D/LConn1
  IGBT-D/RConn2 -- power_losses_diode/LConn1

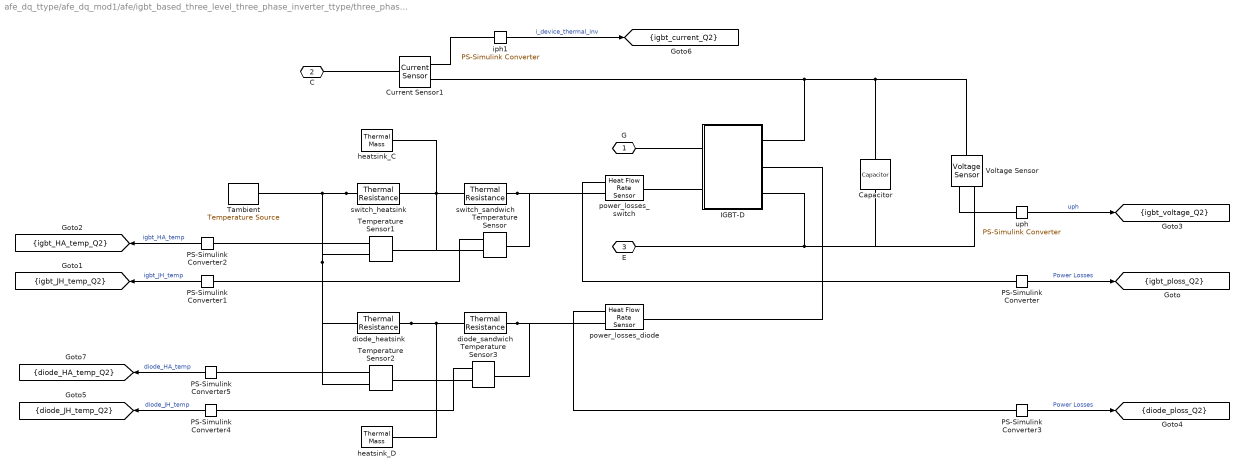
== system afe_dq_ttype/afe_dq_mod1/afe/igbt_based_three_level_three_phase_inverter_ttype/three_phase_inverter_igbt_2th_based_ttype/igbt_thermal_2 ==
  Capacitor : fl_lib/Electrical/Electrical Elements/Capacitor  c=Csnubber_m F  r=Rsnubber_m Ohm  g=0 1/Ohm  i_specify=off  i_priority=None  i=0 A  i_nominal_specify=off  i_nominal_value=1  i_nominal_unit=A  v_specify=off  v_priority=None  v=0 V  v_nominal_specify=off  v_nominal_value=1  v_nominal_unit=V  vc_specify=off  vc_priority=High  vc=0 V  vc_nominal_specify=off  vc_nominal_value=1  vc_nominal_unit=V
  Current Sensor1 : fl_lib/Electrical/Electrical Sensors/Current Sensor
  IGBT-D : Subsystem
  PS-Simulink Converter : nesl_utility/PS-Simulink Converter  PhysicalDomain=network_engine_domain  SubClassName=ps_output  LeftPortType=input  RightPortType=output  PseudoPeriodic=off  Frequencies=[]  VectorFormat=1-D array  Unit=W  AffineConversion=off
  PS-Simulink Converter{1..2,4..5} (4 alike) : nesl_utility/PS-Simulink Converter  PhysicalDomain=network_engine_domain  SubClassName=ps_output  LeftPortType=input  RightPortType=output  PseudoPeriodic=off  Frequencies=[]  VectorFormat=1-D array  Unit=degC  AffineConversion=off
  PS-Simulink Converter3 : nesl_utility/PS-Simulink Converter  PhysicalDomain=network_engine_domain  SubClassName=ps_output  LeftPortType=input  RightPortType=output  PseudoPeriodic=off  Frequencies=[]  VectorFormat=1-D array  Unit=W  AffineConversion=off
  Tambient : fl_lib/Thermal/Thermal Sources/Temperature Source  temperature=Tambient_m degC
  Temperature Sensor{,1..3} (4 alike) : fl_lib/Thermal/Thermal Sensors/Temperature Sensor  temperature_measure=foundation.enum.MeasurementReference.difference
  Voltage Sensor : fl_lib/Electrical/Electrical Sensors/Voltage Sensor
  diode_heatsink : fl_lib/Thermal/Thermal Elements/Thermal Resistance  resistance=rth_diode_HA_m K/W  T_specify=off  T_priority=High  T=0 deltadegC  T_nominal_specify=off  T_nominal_value=1  T_nominal_unit=K  Q_specify=off  Q_priority=None  Q=0 W  Q_nominal_specify=off  Q_nominal_value=1  Q_nominal_unit=W
  diode_sandwich : fl_lib/Thermal/Thermal Elements/Thermal Resistance  resistance=rth_diode_JH_m K/W  T_specify=off  T_priority=High  T=0 degC  T_nominal_specify=off  T_nominal_value=1  T_nominal_unit=K  Q_specify=off  Q_priority=None  Q=0 W  Q_nominal_specify=off  Q_nominal_value=1  Q_nominal_unit=W
  heatsink_C : fl_lib/Thermal/Thermal Elements/Thermal Mass  mass_type=foundation.enum.constant_variable.constant  mass=mass_heatsink_m kg  sp_heat=specific_heat_m J/(K*kg)  mass_min=1e-6 kg  num_ports=foundation.enum.numPorts2.one  m_specify=off  m_priority=High  m=1 kg  m_nominal_specify=off  m_nominal_value=1  m_nominal_unit=kg  T_specify=on  T_priority=High  T=DThs_init_m+Tambient_m degC  T_nominal_specify=off  T_nominal_value=1  T_nominal_unit=K  Q_specify=off  Q_priority=High  Q=0 W  Q_nominal_specify=off  Q_nominal_value=1  Q_nominal_unit=W
  heatsink_D : fl_lib/Thermal/Thermal Elements/Thermal Mass  mass_type=foundation.enum.constant_variable.constant  mass=mass_heatsink_m kg  sp_heat=specific_heat_m J/(K*kg)  mass_min=1e-6 kg  num_ports=foundation.enum.numPorts2.one  m_specify=off  m_priority=High  m=1 kg  m_nominal_specify=off  m_nominal_value=1  m_nominal_unit=kg  T_specify=on  T_priority=High  T=DThs_init_m+Tambient_m degC  T_nominal_specify=off  T_nominal_value=1  T_nominal_unit=K  Q_specify=off  Q_priority=High  Q=0 W  Q_nominal_specify=off  Q_nominal_value=1  Q_nominal_unit=W
  iph1 : nesl_utility/PS-Simulink Converter  PhysicalDomain=network_engine_domain  SubClassName=ps_output  LeftPortType=input  RightPortType=output  PseudoPeriodic=off  Frequencies=[]  VectorFormat=1-D array  Unit=A  AffineConversion=off
  power_losses_diode : fl_lib/Thermal/Thermal Sensors/Heat Flow Rate Sensor
  power_losses_switch : fl_lib/Thermal/Thermal Sensors/Heat Flow Rate Sensor
  switch_heatsink : fl_lib/Thermal/Thermal Elements/Thermal Resistance  resistance=rth_switch_HA_m K/W  T_specify=off  T_priority=High  T=0 deltadegC  T_nominal_specify=off  T_nominal_value=1  T_nominal_unit=K  Q_specify=off  Q_priority=None  Q=0 W  Q_nominal_specify=off  Q_nominal_value=1  Q_nominal_unit=W
  switch_sandwich : fl_lib/Thermal/Thermal Elements/Thermal Resistance  resistance=rth_switch_JH_m K/W  T_specify=off  T_priority=High  T=0 degC  T_nominal_specify=off  T_nominal_value=1  T_nominal_unit=K  Q_specify=off  Q_priority=None  Q=0 W  Q_nominal_specify=off  Q_nominal_value=1  Q_nominal_unit=W
  uph : nesl_utility/PS-Simulink Converter  PhysicalDomain=network_engine_domain  SubClassName=ps_output  LeftPortType=input  RightPortType=output  PseudoPeriodic=off  Frequencies=[]  VectorFormat=1-D array  Unit=V  AffineConversion=off
  G : PMIOPort  Side=Left
  C : PMIOPort  Port=2  Side=Left
  E : PMIOPort  Port=3  Side=Right
  tag scope: diode_HA_temp_Q2=scoped, diode_JH_temp_Q2=scoped, diode_ploss_Q2=scoped, igbt_HA_temp_Q2=scoped, igbt_JH_temp_Q2=scoped, igbt_current_Q2=scoped, igbt_ploss_Q2=scoped, igbt_voltage_Q2=scoped
  wires:
  PS-Simulink Converter5/1 -> [diode_HA_temp_Q2]  "diode_HA_temp"
  PS-Simulink Converter4/1 -> [diode_JH_temp_Q2]  "diode_JH_temp"
  PS-Simulink Converter3/1 -> [diode_ploss_Q2]  "Power Losses"
  uph/1 -> [igbt_voltage_Q2]  "uph"
  iph1/1 -> [igbt_current_Q2]  "i_device_thermal_inv"
  PS-Simulink Converter1/1 -> [igbt_JH_temp_Q2]  "igbt_JH_temp"
  PS-Simulink Converter2/1 -> [igbt_HA_temp_Q2]  "igbt_HA_temp"
  PS-Simulink Converter/1 -> [igbt_ploss_Q2]  "Power Losses"
  connections:
  Temperature Sensor3/RConn2 -- PS-Simulink Converter4/LConn1
  Temperature Sensor2/RConn2 -- PS-Simulink Converter5/LConn1
  power_losses_diode/RConn1 -- PS-Simulink Converter3/LConn1
  diode_heatsink/LConn1 -- diode_sandwich/RConn1 -- Temperature Sensor3/RConn1 -- Temperature Sensor2/LConn1 -- heatsink_D/LConn1
  diode_sandwich/LConn1 -- Temperature Sensor3/LConn1 -- power_losses_diode/RConn2
  Voltage Sensor/RConn1 -- uph/LConn1
  Current Sensor1/RConn1 -- iph1/LConn1
  Current Sensor1/RConn2 -- IGBT-D/RConn1 -- Voltage Sensor/LConn1 -- Capacitor/LConn1
  Current Sensor1/LConn1 -- C/RConn1
  Temperature Sensor1/RConn2 -- PS-Simulink Converter2/LConn1
  switch_heatsink/RConn1 -- Tambient/LConn1 -- Temperature Sensor1/RConn1 -- Temperature Sensor2/RConn1 -- diode_heatsink/RConn1
  Temperature Sensor/RConn2 -- PS-Simulink Converter1/LConn1
  heatsink_C/LConn1 -- switch_heatsink/LConn1 -- switch_sandwich/RConn1 -- Temperature Sensor/RConn1 -- Temperature Sensor1/LConn1
  switch_sandwich/LConn1 -- power_losses_switch/RConn2 -- Temperature Sensor/LConn1
  PS-Simulink Converter/LConn1 -- power_losses_switch/RConn1
  Capacitor/RConn1 -- Voltage Sensor/RConn2 -- IGBT-D/RConn3 -- E/RConn1
  IGBT-D/LConn2 -- power_losses_switch/LConn1
  G/RConn1 -- IGBT-D/LConn1
  IGBT-D/RConn2 -- power_losses_diode/LConn1

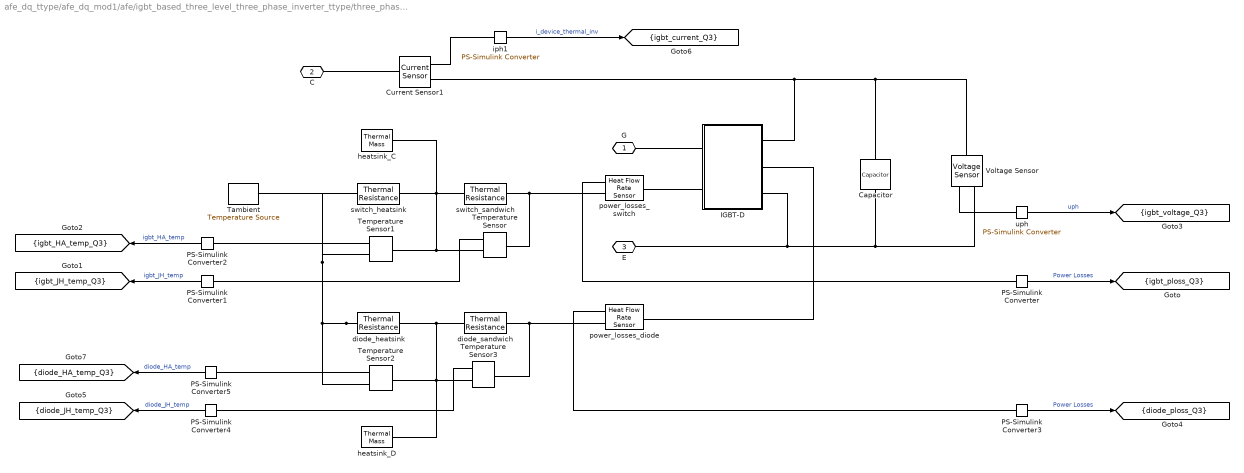
== system afe_dq_ttype/afe_dq_mod1/afe/igbt_based_three_level_three_phase_inverter_ttype/three_phase_inverter_igbt_2th_based_ttype/igbt_thermal_3 ==
  Capacitor : fl_lib/Electrical/Electrical Elements/Capacitor  c=Csnubber_m F  r=Rsnubber_m Ohm  g=0 1/Ohm  i_specify=off  i_priority=None  i=0 A  i_nominal_specify=off  i_nominal_value=1  i_nominal_unit=A  v_specify=off  v_priority=None  v=0 V  v_nominal_specify=off  v_nominal_value=1  v_nominal_unit=V  vc_specify=off  vc_priority=High  vc=0 V  vc_nominal_specify=off  vc_nominal_value=1  vc_nominal_unit=V
  Current Sensor1 : fl_lib/Electrical/Electrical Sensors/Current Sensor
  IGBT-D : Subsystem
  PS-Simulink Converter : nesl_utility/PS-Simulink Converter  PhysicalDomain=network_engine_domain  SubClassName=ps_output  LeftPortType=input  RightPortType=output  PseudoPeriodic=off  Frequencies=[]  VectorFormat=1-D array  Unit=W  AffineConversion=off
  PS-Simulink Converter{1..2,4..5} (4 alike) : nesl_utility/PS-Simulink Converter  PhysicalDomain=network_engine_domain  SubClassName=ps_output  LeftPortType=input  RightPortType=output  PseudoPeriodic=off  Frequencies=[]  VectorFormat=1-D array  Unit=degC  AffineConversion=off
  PS-Simulink Converter3 : nesl_utility/PS-Simulink Converter  PhysicalDomain=network_engine_domain  SubClassName=ps_output  LeftPortType=input  RightPortType=output  PseudoPeriodic=off  Frequencies=[]  VectorFormat=1-D array  Unit=W  AffineConversion=off
  Tambient : fl_lib/Thermal/Thermal Sources/Temperature Source  temperature=Tambient_m degC
  Temperature Sensor{,1..3} (4 alike) : fl_lib/Thermal/Thermal Sensors/Temperature Sensor  temperature_measure=foundation.enum.MeasurementReference.difference
  Voltage Sensor : fl_lib/Electrical/Electrical Sensors/Voltage Sensor
  diode_heatsink : fl_lib/Thermal/Thermal Elements/Thermal Resistance  resistance=rth_diode_HA_m K/W  T_specify=off  T_priority=High  T=0 deltadegC  T_nominal_specify=off  T_nominal_value=1  T_nominal_unit=K  Q_specify=off  Q_priority=None  Q=0 W  Q_nominal_specify=off  Q_nominal_value=1  Q_nominal_unit=W
  diode_sandwich : fl_lib/Thermal/Thermal Elements/Thermal Resistance  resistance=rth_diode_JH_m K/W  T_specify=off  T_priority=High  T=0 degC  T_nominal_specify=off  T_nominal_value=1  T_nominal_unit=K  Q_specify=off  Q_priority=None  Q=0 W  Q_nominal_specify=off  Q_nominal_value=1  Q_nominal_unit=W
  heatsink_C : fl_lib/Thermal/Thermal Elements/Thermal Mass  mass_type=foundation.enum.constant_variable.constant  mass=mass_heatsink_m kg  sp_heat=specific_heat_m J/(K*kg)  mass_min=1e-6 kg  num_ports=foundation.enum.numPorts2.one  m_specify=off  m_priority=High  m=1 kg  m_nominal_specify=off  m_nominal_value=1  m_nominal_unit=kg  T_specify=on  T_priority=High  T=DThs_init_m+Tambient_m degC  T_nominal_specify=off  T_nominal_value=1  T_nominal_unit=K  Q_specify=off  Q_priority=High  Q=0 W  Q_nominal_specify=off  Q_nominal_value=1  Q_nominal_unit=W
  heatsink_D : fl_lib/Thermal/Thermal Elements/Thermal Mass  mass_type=foundation.enum.constant_variable.constant  mass=mass_heatsink_m kg  sp_heat=specific_heat_m J/(K*kg)  mass_min=1e-6 kg  num_ports=foundation.enum.numPorts2.one  m_specify=off  m_priority=High  m=1 kg  m_nominal_specify=off  m_nominal_value=1  m_nominal_unit=kg  T_specify=on  T_priority=High  T=DThs_init_m+Tambient_m degC  T_nominal_specify=off  T_nominal_value=1  T_nominal_unit=K  Q_specify=off  Q_priority=High  Q=0 W  Q_nominal_specify=off  Q_nominal_value=1  Q_nominal_unit=W
  iph1 : nesl_utility/PS-Simulink Converter  PhysicalDomain=network_engine_domain  SubClassName=ps_output  LeftPortType=input  RightPortType=output  PseudoPeriodic=off  Frequencies=[]  VectorFormat=1-D array  Unit=A  AffineConversion=off
  power_losses_diode : fl_lib/Thermal/Thermal Sensors/Heat Flow Rate Sensor
  power_losses_switch : fl_lib/Thermal/Thermal Sensors/Heat Flow Rate Sensor
  switch_heatsink : fl_lib/Thermal/Thermal Elements/Thermal Resistance  resistance=rth_switch_HA_m K/W  T_specify=off  T_priority=High  T=0 deltadegC  T_nominal_specify=off  T_nominal_value=1  T_nominal_unit=K  Q_specify=off  Q_priority=None  Q=0 W  Q_nominal_specify=off  Q_nominal_value=1  Q_nominal_unit=W
  switch_sandwich : fl_lib/Thermal/Thermal Elements/Thermal Resistance  resistance=rth_switch_JH_m K/W  T_specify=off  T_priority=High  T=0 degC  T_nominal_specify=off  T_nominal_value=1  T_nominal_unit=K  Q_specify=off  Q_priority=None  Q=0 W  Q_nominal_specify=off  Q_nominal_value=1  Q_nominal_unit=W
  uph : nesl_utility/PS-Simulink Converter  PhysicalDomain=network_engine_domain  SubClassName=ps_output  LeftPortType=input  RightPortType=output  PseudoPeriodic=off  Frequencies=[]  VectorFormat=1-D array  Unit=V  AffineConversion=off
  G : PMIOPort  Side=Left
  C : PMIOPort  Port=2  Side=Left
  E : PMIOPort  Port=3  Side=Right
  tag scope: diode_HA_temp_Q3=scoped, diode_JH_temp_Q3=scoped, diode_ploss_Q3=scoped, igbt_HA_temp_Q3=scoped, igbt_JH_temp_Q3=scoped, igbt_current_Q3=scoped, igbt_ploss_Q3=scoped, igbt_voltage_Q3=scoped
  wires:
  PS-Simulink Converter/1 -> [igbt_ploss_Q3]  "Power Losses"
  PS-Simulink Converter2/1 -> [igbt_HA_temp_Q3]  "igbt_HA_temp"
  PS-Simulink Converter1/1 -> [igbt_JH_temp_Q3]  "igbt_JH_temp"
  iph1/1 -> [igbt_current_Q3]  "i_device_thermal_inv"
  uph/1 -> [igbt_voltage_Q3]  "uph"
  PS-Simulink Converter3/1 -> [diode_ploss_Q3]  "Power Losses"
  PS-Simulink Converter4/1 -> [diode_JH_temp_Q3]  "diode_JH_temp"
  PS-Simulink Converter5/1 -> [diode_HA_temp_Q3]  "diode_HA_temp"
  connections:
  Voltage Sensor/RConn2 -- Capacitor/RConn1 -- IGBT-D/RConn3 -- E/RConn1
  PS-Simulink Converter/LConn1 -- power_losses_switch/RConn1
  Temperature Sensor/LConn1 -- power_losses_switch/RConn2 -- switch_sandwich/LConn1
  Temperature Sensor1/LConn1 -- Temperature Sensor/RConn1 -- switch_sandwich/RConn1 -- switch_heatsink/LConn1 -- heatsink_C/LConn1
  Temperature Sensor/RConn2 -- PS-Simulink Converter1/LConn1
  diode_heatsink/RConn1 -- Temperature Sensor2/RConn1 -- Temperature Sensor1/RConn1 -- Tambient/LConn1 -- switch_heatsink/RConn1
  Temperature Sensor1/RConn2 -- PS-Simulink Converter2/LConn1
  Current Sensor1/LConn1 -- C/RConn1
  Capacitor/LConn1 -- Voltage Sensor/LConn1 -- IGBT-D/RConn1 -- Current Sensor1/RConn2
  Current Sensor1/RConn1 -- iph1/LConn1
  Voltage Sensor/RConn1 -- uph/LConn1
  power_losses_diode/RConn2 -- Temperature Sensor3/LConn1 -- diode_sandwich/LConn1
  heatsink_D/LConn1 -- Temperature Sensor2/LConn1 -- Temperature Sensor3/RConn1 -- diode_sandwich/RConn1 -- diode_heatsink/LConn1
  power_losses_diode/RConn1 -- PS-Simulink Converter3/LConn1
  Temperature Sensor2/RConn2 -- PS-Simulink Converter5/LConn1
  Temperature Sensor3/RConn2 -- PS-Simulink Converter4/LConn1
  IGBT-D/LConn2 -- power_losses_switch/LConn1
  G/RConn1 -- IGBT-D/LConn1
  IGBT-D/RConn2 -- power_losses_diode/LConn1
